simulink library "utils"  (R2024b)
settings: Solver=VariableStepAuto  StartTime=0.0  StopTime=10.0  RelTol=1e-3
undefined symbols (not defined in the file): plane
settings Model: Creator=domac  LastModifiedBy=domac

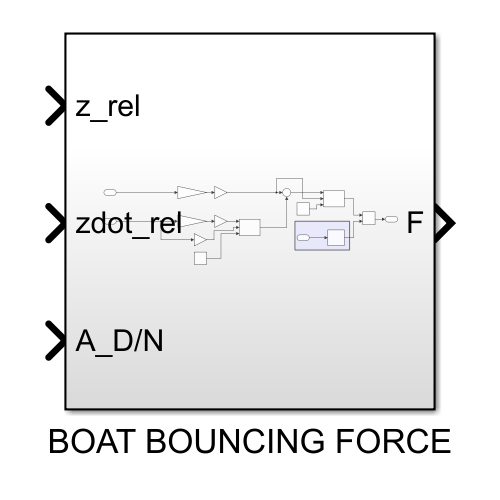
[thumbnail: Simulink's stored preview of the top-level diagram]
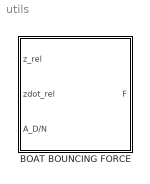
== system utils ==
  BOAT BOUNCING FORCE : Subsystem

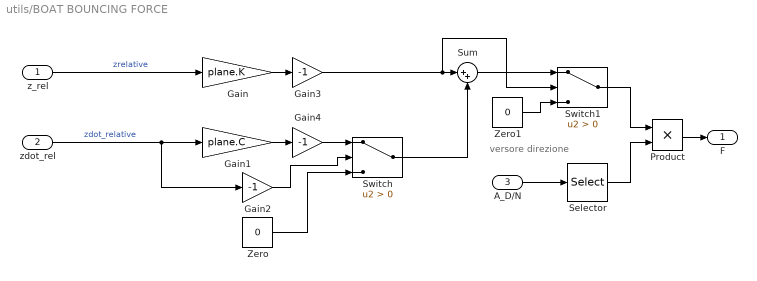
== system utils/BOAT BOUNCING FORCE ==
  note: versore direzione
  z_rel : Inport
  zdot_rel : Inport  Port=2
  A_D/N : Inport  Port=3
  Gain : Gain  Gain=plane.K
  Gain1 : Gain  Gain=plane.C
  Gain2 : Gain  Gain=-1
  Gain3 : Gain  Gain=-1
  Gain4 : Gain  Gain=-1
  Product : Product
  Selector : Selector  NumberOfDimensions=2  InputPortWidth=3  IndexOptions=Index vector (dialog),Index vector (dialog)  Indices=1,[1, 2, 3]  OutputSizes=1,1
  Sum : Sum  Inputs=|++
  Switch : Switch  Criteria=u2 > Threshold  SaturateOnIntegerOverflow=off  InputSameDT=off
  Switch1 : Switch  Criteria=u2 > Threshold  SaturateOnIntegerOverflow=off  InputSameDT=off
  Zero : Constant  Value=0  OutDataTypeStr=Inherit: Inherit via back propagation
  Zero1 : Constant  Value=0  OutDataTypeStr=Inherit: Inherit via back propagation
  F : Outport
  wires:
  Zero/1 -> Switch/3
  Gain3/1 -> Switch1/2, Sum/1
  Gain4/1 -> Switch/1
  Zero1/1 -> Switch1/3
  Switch/1 -> Sum/2
  Gain/1 -> Gain3/1
  Sum/1 -> Switch1/1
  zdot_rel/1 -> Gain2/1, Gain1/1  "zdot_relative"
  Gain1/1 -> Gain4/1
  Gain2/1 -> Switch/2
  z_rel/1 -> Gain/1  "zrelative"
  A_D/N/1 -> Selector/1
  Switch1/1 -> Product/1
  Selector/1 -> Product/2
  Product/1 -> F/1
